simulink model "sma_nonlinear_closed_loop"  (R2023b)
settings: Solver=VariableStepAuto  StartTime=0.0  StopTime=10.0  RelTol=1e-3
values from neighbouring files (symbols this model uses):
  beta = 1.5    [sma_cascade_control.m]
  Cth = 25.1e-3    (= 0.0251)    [sma_cascade_control.m]
  Kmax = 3.92e3    (= 3920)    [sma_cascade_control.m]
  l = 15e-2    (= 0.15)    [sma_cascade_control.m]
  Le = 55e-3    (= 0.055)    [sma_cascade_control.m]
  m = 15e-3    (= 0.015)    [sma_cascade_control.m]
  m_eq = J/r2 + m*r2    (= 0.00511944444444)    [sma_cascade_control.m]
  r1 = 0.45e-2    (= 0.0045)    [sma_cascade_control.m]
  r2 = 4.5e-2    (= 0.045)    [sma_cascade_control.m]
  Ramb = 1/(h*pi*d*l)    (= 1619.89763961)    [sma_cascade_control.m]
  Re = 4.8    [sma_cascade_control.m]
  rho = r2/r1    (= 10)    [sma_cascade_control.m]
  Rth = 16.7    [sma_cascade_control.m]
  T0 = 273.15    [sma_cascade_control.m]
  Tamb = 24 + T0    (= 297.15)    [sma_cascade_control.m]
  Tavg = 70    [sma_cascade_control.m]
  Tdiff = 20    [sma_cascade_control.m]
  Tp = 15 + T0    (= 288.15)    [sma_cascade_control.m]
  u_eq = Re*x1_eq    [sma_cascade_control.m]
  x1_eq = sqrt((1/Re)*(h*S*(x2_eq_k - Tamb) + (1/Rth)*(x2_eq_k - Tp)))    [sma_cascade_control.m]
  x2_eq_k = x2_eq + T0    [sma_cascade_control.m]
  x3_eq = 4e-2    (= 0.04)    [sma_cascade_control.m]
  x4_eq = 0    [sma_cascade_control.m]
undefined symbols (not defined in the file or in its folder): A1, A2, B1, B2, C1, C2, D1, D2, magnitude
settings Model: Creator=Utente  LastModifiedBy=Utente

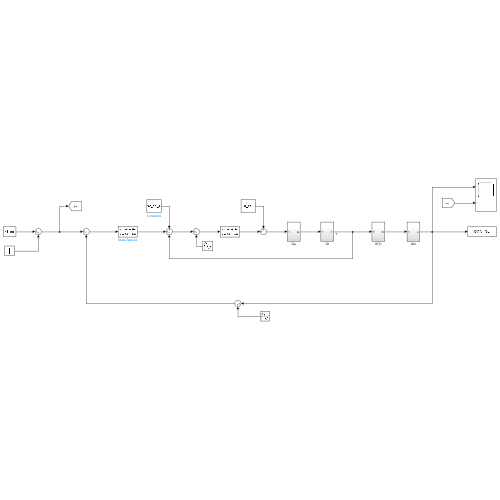
[thumbnail: Simulink's stored preview of the top-level diagram]
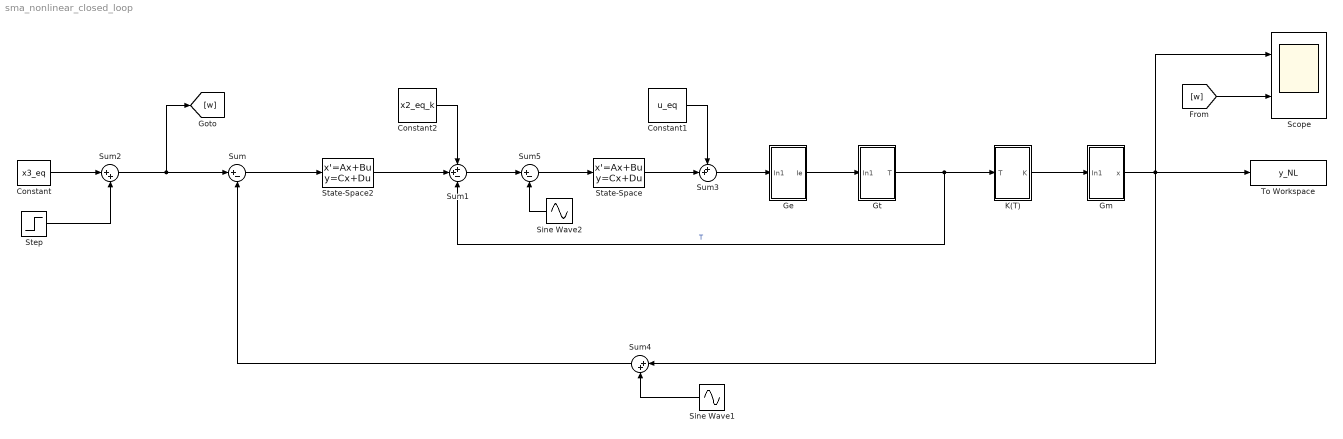
== system sma_nonlinear_closed_loop ==
  Constant : Constant  Value=x3_eq
  Constant1 : Constant  Value=u_eq
  Constant2 : Constant  Value=x2_eq_k
  Ge : Subsystem
  Gm : Subsystem
  Gt : Subsystem
  K(T) : Subsystem
  Scope : Scope  NumInputPorts=2
  Sine Wave1 : Sin  Amplitude=5e-4  Frequency=20  SampleTime=0
  Sine Wave2 : Sin  Frequency=2e4  SampleTime=0
  State-Space : StateSpace  A=A1  B=B1  C=C1  D=D1  InitialCondition=0
  State-Space2 : StateSpace  A=A2  B=B2  C=C2  D=D2  InitialCondition=0
  Step : Step  After=0.005  SampleTime=0
  Sum : Sum  Inputs=|+-
  Sum1 : Sum  Inputs=++-
  Sum2 : Sum  Inputs=|++
  Sum3 : Sum  Inputs=++|
  Sum4 : Sum  Inputs=|++
  Sum5 : Sum  Inputs=|+-
  To Workspace : ToWorkspace  VariableName=y_NL  SaveFormat=Timeseries  SampleTime=-1
  wires:
  Sum1/1 -> Sum5/1
  Sum5/1 -> State-Space/1
  State-Space2/1 -> Sum1/2
  Sum/1 -> State-Space2/1
  Sum4/1 -> Sum/2
  Sine Wave1/1 -> Sum4/2
  Sum2/1 -> [w], Sum/1
  K(T)/1(K) -> Gm/1(In1)
  Gt/1(T) -> K(T)/1(T), Sum1/3  "T"
  Sine Wave2/1 -> Sum5/2
  Ge/1(Ie) -> Gt/1(In1)
  Gm/1(x) -> Scope/1, Sum4/1, To Workspace/1
  Constant/1 -> Sum2/1
  Step/1 -> Sum2/2
  Constant2/1 -> Sum1/1
  [w] -> Scope/2
  State-Space/1 -> Sum3/2
  Sum3/1 -> Ge/1(In1)
  Constant1/1 -> Sum3/1

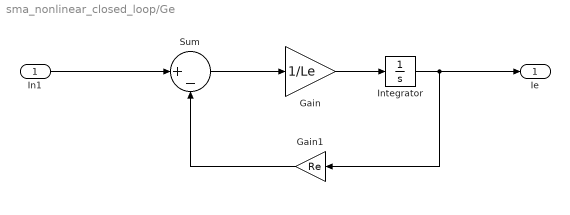
== system sma_nonlinear_closed_loop/Ge ==
  In1 : Inport
  Gain : Gain  Gain=1/Le
  Gain1 : Gain  Gain=Re
  Integrator : Integrator  InitialCondition=x1_eq
  Sum : Sum  Inputs=|+-
  Ie : Outport
  wires:
  Integrator/1 -> Ie/1, Gain1/1
  Gain1/1 -> Sum/2
  Sum/1 -> Gain/1
  In1/1 -> Sum/1
  Gain/1 -> Integrator/1

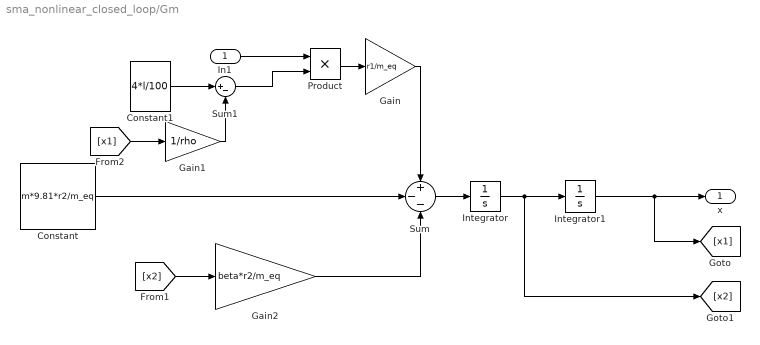
== system sma_nonlinear_closed_loop/Gm ==
  In1 : Inport
  Constant : Constant  Value=m*9.81*r2/m_eq
  Constant1 : Constant  Value=4*l/100
  Gain : Gain  Gain=r1/m_eq
  Gain1 : Gain  Gain=1/rho
  Gain2 : Gain  Gain=beta*r2/m_eq
  Integrator : Integrator  InitialCondition=x4_eq
  Integrator1 : Integrator  InitialCondition=x3_eq  LimitOutput=on  UpperSaturationLimit=0.16  LowerSaturationLimit=0
  Product : Product
  Sum : Sum  Inputs=+--
  Sum1 : Sum  Inputs=|+-
  x : Outport
  wires:
  In1/1 -> Product/1
  Integrator/1 -> [x2], Integrator1/1
  Integrator1/1 -> [x1], x/1
  [x2] -> Gain2/1
  Gain2/1 -> Sum/3
  Constant1/1 -> Sum1/1
  Sum1/1 -> Product/2
  Product/1 -> Gain/1
  Gain/1 -> Sum/1
  Constant/1 -> Sum/2
  Sum/1 -> Integrator/1
  [x1] -> Gain1/1
  Gain1/1 -> Sum1/2

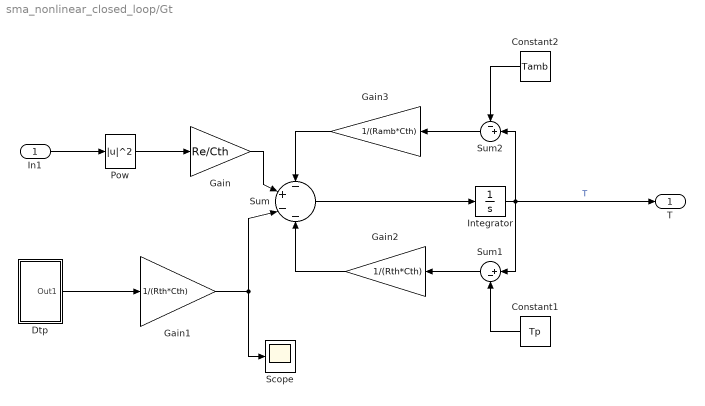
== system sma_nonlinear_closed_loop/Gt ==
  In1 : Inport
  Constant1 : Constant  Value=Tp
  Constant2 : Constant  Value=Tamb
  Dtp : Subsystem
  Gain : Gain  Gain=Re/Cth
  Gain1 : Gain  Gain=1/(Rth*Cth)
  Gain2 : Gain  Gain=1/(Rth*Cth)
  Gain3 : Gain  Gain=1/(Ramb*Cth)
  Integrator : Integrator  InitialCondition=x2_eq_k
  Pow : Math  Operator=magnitude^2  SignedPower=on  RndMeth=Zero
  Scope : Scope
  Sum : Sum  Inputs=-+--
  Sum1 : Sum  Inputs=|+-
  Sum2 : Sum  Inputs=-+|
  T : Outport
  wires:
  Sum2/1 -> Gain3/1
  Constant1/1 -> Sum1/2
  Integrator/1 -> T/1, Sum2/2, Sum1/1  "T"
  Sum/1 -> Integrator/1
  Gain/1 -> Sum/2
  Sum1/1 -> Gain2/1
  Pow/1 -> Gain/1
  Constant2/1 -> Sum2/1
  Gain3/1 -> Sum/1
  In1/1 -> Pow/1
  Dtp/1(Out1) -> Gain1/1
  Gain2/1 -> Sum/4
  Gain1/1 -> Sum/3, Scope/1

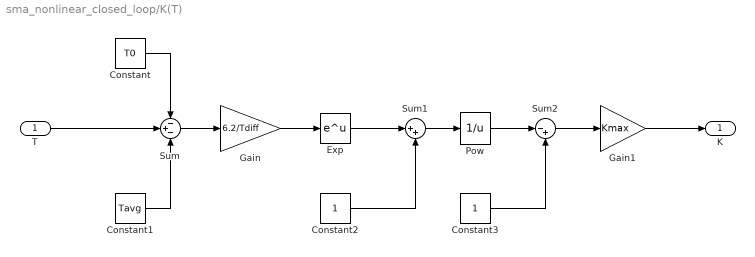
== system sma_nonlinear_closed_loop/K(T) ==
  T : Inport
  Constant : Constant  Value=T0
  Constant1 : Constant  Value=Tavg
  Constant2 : Constant
  Constant3 : Constant
  Exp : Math
  Gain : Gain  Gain=6.2/Tdiff
  Gain1 : Gain  Gain=Kmax
  Pow : Math  Operator=reciprocal  SignedPower=on  RndMeth=Zero
  Sum : Sum  Inputs=-+-
  Sum1 : Sum  Inputs=|++
  Sum2 : Sum  Inputs=|-+
  K : Outport
  wires:
  Constant3/1 -> Sum2/2
  Sum1/1 -> Pow/1
  Pow/1 -> Sum2/1
  Sum2/1 -> Gain1/1
  Exp/1 -> Sum1/1
  Constant2/1 -> Sum1/2
  Gain/1 -> Exp/1
  Sum/1 -> Gain/1
  Gain1/1 -> K/1
  T/1 -> Sum/2
  Constant1/1 -> Sum/3
  Constant/1 -> Sum/1

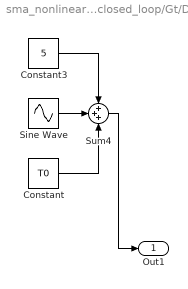
== system sma_nonlinear_closed_loop/Gt/Dtp ==
  Constant : Constant  Value=T0
  Constant3 : Constant  Value=5
  Sine Wave : Sin  Amplitude=5  Frequency=5  SampleTime=0
  Sum4 : Sum  Inputs=+++
  Out1 : Outport
  wires:
  Sum4/1 -> Out1/1
  Sine Wave/1 -> Sum4/2
  Constant3/1 -> Sum4/1
  Constant/1 -> Sum4/3
